simulink model "generic_src"  (Simulink 10.3)
settings: Solver=ode45  StartTime=0.0  StopTime=inf  RelTol=1e-3  EnableMultiTasking=on
undefined symbols (not defined in the file or in its folder): Area_Front, Area_Rear, ay_max_off, ay_max_on, ay_per_mu_max_off, ay_per_mu_max_on, Brake_ratio, brake_valve_ctrl_kP, cat1mode1_higher, cat1mode1_lower, cat1mode2_higher, cat1mode2_lower, cat1mode3_higher, cat1mode3_lower, cat2mode1_higher, cat2mode1_lower, cat2mode2_higher, cat2mode2_lower, cat2mode3_higher, cat2mode3_lower, delta_vel, diff_lock_fac, diff_lock_off, diff_lock_on, ESP_ctrl_kD, ESP_ctrl_kI, ESP_ctrl_kP, ESP_ctrl_restore_kI, ESP_min_throttle_fac, f_ax, f_slip, g, higherlimit_highvel, higherlimit_lowvel, highervel_fac, highervelocity_fac, InitialConditionForIntegrator, limit_acc, limit_selectlow, limit_starting, limit_vdiff, locktime_throttle, lowerlimit_highvel, lowerlimit_lowvel, lowervel_fac, lowervelocity_fac, min_throttle, MPS2KMPH, MSR_ctrl_kD, MSR_ctrl_kI, MSR_ctrl_kP, MSR_min_throttle_fac, PID_kP_sideslip, PID_kP_yawrate, RADpS2RpM, rBrake, RpM2RADpS, SH_SL_switch, sideslip_vel_corr, sidesplip_deviation_max ... (+35)
libraries: CarMaker4SL x136, simulink x55, simulink_extras x6
(part 5 of 9)

== system generic_src/CarMaker/IPG Vehicle/PowerTrain/PTControl Example/PTControl_In/CreateBus PTC BatteryLVIn ==
  In : Inport
  BusCreator : BusCreator  Inputs=8
  Demux : Demux  Outputs=8
      settings: DisplayOption=none
  Out : Outport  VectorParamsAs1DForOutWhenUnconnected=off
  wires:
  Demux/7 -> BusCreator/7  "PTC BattLVIn Temp"
  In/1 -> Demux/1
  Demux/8 -> BusCreator/8  "PTC BattLVIn TempCool_out"
  Demux/6 -> BusCreator/6  "PTC BattLVIn Pwr_max"
  Demux/1 -> BusCreator/1  "PTC BattLVIn SOC"
  Demux/3 -> BusCreator/3  "PTC BattLVIn Current"
  Demux/2 -> BusCreator/2  "PTC BattLVIn SOH"
  BusCreator/1 -> Out/1
  Demux/4 -> BusCreator/4  "PTC BattLVIn AOC"
  Demux/5 -> BusCreator/5  "PTC BattLVIn Energy"

== system generic_src/CarMaker/IPG Vehicle/PowerTrain/PTControl Example/PTControl_In/CreateBus PTC ClutchIn0 ==
  In : Inport
  BusCreator : BusCreator  Inputs=6
  Demux : Demux  Outputs=6
      settings: DisplayOption=none
  Out : Outport  VectorParamsAs1DForOutWhenUnconnected=off
  wires:
  Demux/6 -> BusCreator/6  "PTC ClutchIn0 i_TrqIn2Out"
  Demux/5 -> BusCreator/5  "PTC ClutchIn0 Trq_out"
  Demux/4 -> BusCreator/4  "PTC ClutchIn0 Trq_in"
  Demux/3 -> BusCreator/3  "PTC ClutchIn0 rotv_out"
  Demux/2 -> BusCreator/2  "PTC ClutchIn0 rotv_in"
  Demux/1 -> BusCreator/1  "PTC ClutchIn0 Pos"
  BusCreator/1 -> Out/1
  In/1 -> Demux/1

== system generic_src/CarMaker/IPG Vehicle/PowerTrain/PTControl Example/PTControl_In/CreateBus PTC ClutchIn1 ==
  In : Inport
  BusCreator : BusCreator  Inputs=6
  Demux : Demux  Outputs=6
      settings: DisplayOption=none
  Out : Outport  VectorParamsAs1DForOutWhenUnconnected=off
  wires:
  Demux/6 -> BusCreator/6  "PTC ClutchIn1 i_TrqIn2Out"
  Demux/5 -> BusCreator/5  "PTC ClutchIn1 Trq_out"
  Demux/4 -> BusCreator/4  "PTC ClutchIn1 Trq_in"
  Demux/3 -> BusCreator/3  "PTC ClutchIn1 rotv_out"
  Demux/2 -> BusCreator/2  "PTC ClutchIn1 rotv_in"
  Demux/1 -> BusCreator/1  "PTC ClutchIn1 Pos"
  BusCreator/1 -> Out/1
  In/1 -> Demux/1

== system generic_src/CarMaker/IPG Vehicle/PowerTrain/PTControl Example/PTControl_In/CreateBus PTC ClutchIn10 ==
  In : Inport
  BusCreator : BusCreator  Inputs=6
  Demux : Demux  Outputs=6
      settings: DisplayOption=none
  Out : Outport  VectorParamsAs1DForOutWhenUnconnected=off
  wires:
  Demux/6 -> BusCreator/6  "PTC ClutchIn10 i_TrqIn2Out"
  Demux/5 -> BusCreator/5  "PTC ClutchIn10 Trq_out"
  Demux/4 -> BusCreator/4  "PTC ClutchIn10 Trq_in"
  Demux/3 -> BusCreator/3  "PTC ClutchIn10 rotv_out"
  Demux/2 -> BusCreator/2  "PTC ClutchIn10 rotv_in"
  Demux/1 -> BusCreator/1  "PTC ClutchIn10 Pos"
  BusCreator/1 -> Out/1
  In/1 -> Demux/1

== system generic_src/CarMaker/IPG Vehicle/PowerTrain/PTControl Example/PTControl_In/CreateBus PTC ClutchIn11 ==
  In : Inport
  BusCreator : BusCreator  Inputs=6
  Demux : Demux  Outputs=6
      settings: DisplayOption=none
  Out : Outport  VectorParamsAs1DForOutWhenUnconnected=off
  wires:
  Demux/6 -> BusCreator/6  "PTC ClutchIn11 i_TrqIn2Out"
  Demux/5 -> BusCreator/5  "PTC ClutchIn11 Trq_out"
  Demux/4 -> BusCreator/4  "PTC ClutchIn11 Trq_in"
  Demux/3 -> BusCreator/3  "PTC ClutchIn11 rotv_out"
  Demux/2 -> BusCreator/2  "PTC ClutchIn11 rotv_in"
  Demux/1 -> BusCreator/1  "PTC ClutchIn11 Pos"
  BusCreator/1 -> Out/1
  In/1 -> Demux/1

== system generic_src/CarMaker/IPG Vehicle/PowerTrain/PTControl Example/PTControl_In/CreateBus PTC ClutchIn2 ==
  In : Inport
  BusCreator : BusCreator  Inputs=6
  Demux : Demux  Outputs=6
      settings: DisplayOption=none
  Out : Outport  VectorParamsAs1DForOutWhenUnconnected=off
  wires:
  Demux/6 -> BusCreator/6  "PTC ClutchIn2 i_TrqIn2Out"
  Demux/5 -> BusCreator/5  "PTC ClutchIn2 Trq_out"
  Demux/4 -> BusCreator/4  "PTC ClutchIn2 Trq_in"
  Demux/3 -> BusCreator/3  "PTC ClutchIn2 rotv_out"
  Demux/2 -> BusCreator/2  "PTC ClutchIn2 rotv_in"
  Demux/1 -> BusCreator/1  "PTC ClutchIn2 Pos"
  BusCreator/1 -> Out/1
  In/1 -> Demux/1

== system generic_src/CarMaker/IPG Vehicle/PowerTrain/PTControl Example/PTControl_In/CreateBus PTC ClutchIn3 ==
  In : Inport
  BusCreator : BusCreator  Inputs=6
  Demux : Demux  Outputs=6
      settings: DisplayOption=none
  Out : Outport  VectorParamsAs1DForOutWhenUnconnected=off
  wires:
  Demux/6 -> BusCreator/6  "PTC ClutchIn3 i_TrqIn2Out"
  Demux/5 -> BusCreator/5  "PTC ClutchIn3 Trq_out"
  Demux/4 -> BusCreator/4  "PTC ClutchIn3 Trq_in"
  Demux/3 -> BusCreator/3  "PTC ClutchIn3 rotv_out"
  Demux/2 -> BusCreator/2  "PTC ClutchIn3 rotv_in"
  Demux/1 -> BusCreator/1  "PTC ClutchIn3 Pos"
  BusCreator/1 -> Out/1
  In/1 -> Demux/1

== system generic_src/CarMaker/IPG Vehicle/PowerTrain/PTControl Example/PTControl_In/CreateBus PTC ClutchIn4 ==
  In : Inport
  BusCreator : BusCreator  Inputs=6
  Demux : Demux  Outputs=6
      settings: DisplayOption=none
  Out : Outport  VectorParamsAs1DForOutWhenUnconnected=off
  wires:
  Demux/6 -> BusCreator/6  "PTC ClutchIn4 i_TrqIn2Out"
  Demux/5 -> BusCreator/5  "PTC ClutchIn4 Trq_out"
  Demux/4 -> BusCreator/4  "PTC ClutchIn4 Trq_in"
  Demux/3 -> BusCreator/3  "PTC ClutchIn4 rotv_out"
  Demux/2 -> BusCreator/2  "PTC ClutchIn4 rotv_in"
  Demux/1 -> BusCreator/1  "PTC ClutchIn4 Pos"
  BusCreator/1 -> Out/1
  In/1 -> Demux/1

== system generic_src/CarMaker/IPG Vehicle/PowerTrain/PTControl Example/PTControl_In/CreateBus PTC ClutchIn5 ==
  In : Inport
  BusCreator : BusCreator  Inputs=6
  Demux : Demux  Outputs=6
      settings: DisplayOption=none
  Out : Outport  VectorParamsAs1DForOutWhenUnconnected=off
  wires:
  Demux/6 -> BusCreator/6  "PTC ClutchIn5 i_TrqIn2Out"
  Demux/5 -> BusCreator/5  "PTC ClutchIn5 Trq_out"
  Demux/4 -> BusCreator/4  "PTC ClutchIn5 Trq_in"
  Demux/3 -> BusCreator/3  "PTC ClutchIn5 rotv_out"
  Demux/2 -> BusCreator/2  "PTC ClutchIn5 rotv_in"
  Demux/1 -> BusCreator/1  "PTC ClutchIn5 Pos"
  BusCreator/1 -> Out/1
  In/1 -> Demux/1

== system generic_src/CarMaker/IPG Vehicle/PowerTrain/PTControl Example/PTControl_In/CreateBus PTC ClutchIn6 ==
  In : Inport
  BusCreator : BusCreator  Inputs=6
  Demux : Demux  Outputs=6
      settings: DisplayOption=none
  Out : Outport  VectorParamsAs1DForOutWhenUnconnected=off
  wires:
  Demux/6 -> BusCreator/6  "PTC ClutchIn6 i_TrqIn2Out"
  Demux/5 -> BusCreator/5  "PTC ClutchIn6 Trq_out"
  Demux/4 -> BusCreator/4  "PTC ClutchIn6 Trq_in"
  Demux/3 -> BusCreator/3  "PTC ClutchIn6 rotv_out"
  Demux/2 -> BusCreator/2  "PTC ClutchIn6 rotv_in"
  Demux/1 -> BusCreator/1  "PTC ClutchIn6 Pos"
  BusCreator/1 -> Out/1
  In/1 -> Demux/1

== system generic_src/CarMaker/IPG Vehicle/PowerTrain/PTControl Example/PTControl_In/CreateBus PTC ClutchIn7 ==
  In : Inport
  BusCreator : BusCreator  Inputs=6
  Demux : Demux  Outputs=6
      settings: DisplayOption=none
  Out : Outport  VectorParamsAs1DForOutWhenUnconnected=off
  wires:
  Demux/6 -> BusCreator/6  "PTC ClutchIn7 i_TrqIn2Out"
  Demux/5 -> BusCreator/5  "PTC ClutchIn7 Trq_out"
  Demux/4 -> BusCreator/4  "PTC ClutchIn7 Trq_in"
  Demux/3 -> BusCreator/3  "PTC ClutchIn7 rotv_out"
  Demux/2 -> BusCreator/2  "PTC ClutchIn7 rotv_in"
  Demux/1 -> BusCreator/1  "PTC ClutchIn7 Pos"
  BusCreator/1 -> Out/1
  In/1 -> Demux/1

== system generic_src/CarMaker/IPG Vehicle/PowerTrain/PTControl Example/PTControl_In/CreateBus PTC ClutchIn8 ==
  In : Inport
  BusCreator : BusCreator  Inputs=6
  Demux : Demux  Outputs=6
      settings: DisplayOption=none
  Out : Outport  VectorParamsAs1DForOutWhenUnconnected=off
  wires:
  Demux/6 -> BusCreator/6  "PTC ClutchIn8 i_TrqIn2Out"
  Demux/5 -> BusCreator/5  "PTC ClutchIn8 Trq_out"
  Demux/4 -> BusCreator/4  "PTC ClutchIn8 Trq_in"
  Demux/3 -> BusCreator/3  "PTC ClutchIn8 rotv_out"
  Demux/2 -> BusCreator/2  "PTC ClutchIn8 rotv_in"
  Demux/1 -> BusCreator/1  "PTC ClutchIn8 Pos"
  BusCreator/1 -> Out/1
  In/1 -> Demux/1

== system generic_src/CarMaker/IPG Vehicle/PowerTrain/PTControl Example/PTControl_In/CreateBus PTC ClutchIn9 ==
  In : Inport
  BusCreator : BusCreator  Inputs=6
  Demux : Demux  Outputs=6
      settings: DisplayOption=none
  Out : Outport  VectorParamsAs1DForOutWhenUnconnected=off
  wires:
  Demux/6 -> BusCreator/6  "PTC ClutchIn9 i_TrqIn2Out"
  Demux/5 -> BusCreator/5  "PTC ClutchIn9 Trq_out"
  Demux/4 -> BusCreator/4  "PTC ClutchIn9 Trq_in"
  Demux/3 -> BusCreator/3  "PTC ClutchIn9 rotv_out"
  Demux/2 -> BusCreator/2  "PTC ClutchIn9 rotv_in"
  Demux/1 -> BusCreator/1  "PTC ClutchIn9 Pos"
  BusCreator/1 -> Out/1
  In/1 -> Demux/1

== system generic_src/CarMaker/IPG Vehicle/PowerTrain/PTControl Example/PTControl_In/CreateBus PTC Control Units ==
  In : Inport
  BusCreator : BusCreator  Inputs=4
  Demux : Demux
      settings: DisplayOption=none
  Out : Outport  VectorParamsAs1DForOutWhenUnconnected=off
  wires:
  Demux/4 -> BusCreator/4  "PTC BCU_Status"
  Demux/3 -> BusCreator/3  "PTC TCU_Status"
  Demux/2 -> BusCreator/2  "PTC MCU_Status"
  Demux/1 -> BusCreator/1  "PTC ECU_Status"
  BusCreator/1 -> Out/1
  In/1 -> Demux/1

== system generic_src/CarMaker/IPG Vehicle/PowerTrain/PTControl Example/PTControl_In/CreateBus PTC DriveSrcIn ==
  In : Inport
  BusCreator : BusCreator  Inputs=4
  Demux : Demux
      settings: DisplayOption=none
  Out : Outport  VectorParamsAs1DForOutWhenUnconnected=off
  wires:
  Demux/4 -> BusCreator/4  "PTC DriveSrcIn_d3 Trq_DriveSrc_trg"
  Demux/3 -> BusCreator/3  "PTC DriveSrcIn_d2 Trq_DriveSrc_trg"
  Demux/2 -> BusCreator/2  "PTC DriveSrcIn_d1 Trq_DriveSrc_trg"
  Demux/1 -> BusCreator/1  "PTC DriveSrcIn_d0 Trq_DriveSrc_trg"
  BusCreator/1 -> Out/1
  In/1 -> Demux/1

== system generic_src/CarMaker/IPG Vehicle/PowerTrain/PTControl Example/PTControl_In/CreateBus PTC EngineIn ==
  In : Inport
  BusCreator : BusCreator  Inputs=7
  Demux : Demux  Outputs=7
      settings: DisplayOption=none
  Out : Outport  VectorParamsAs1DForOutWhenUnconnected=off
  wires:
  Demux/7 -> BusCreator/7  "PTC EngineIn FuelFlow"
  Demux/6 -> BusCreator/6  "PTC EngineIn TrqOpt"
  Demux/5 -> BusCreator/5  "PTC EngineIn TrqFull"
  Demux/4 -> BusCreator/4  "PTC EngineIn TrqDrag"
  Demux/3 -> BusCreator/3  "PTC EngineIn Trq"
  Demux/2 -> BusCreator/2  "PTC EngineIn rotv"
  Demux/1 -> BusCreator/1  "PTC EngineIn Engine_on"
  BusCreator/1 -> Out/1
  In/1 -> Demux/1

== system generic_src/CarMaker/IPG Vehicle/PowerTrain/PTControl Example/PTControl_In/CreateBus PTC GearboxIn0 ==
  In : Inport
  BusCreator : BusCreator  Inputs=20
  Demux : Demux  Outputs=20
      settings: DisplayOption=none
  Out : Outport  VectorParamsAs1DForOutWhenUnconnected=off
  wires:
  Demux/20 -> BusCreator/20  "PTC GearboxIn0 Clutch_dis i_TrqIn2Out"
  Demux/19 -> BusCreator/19  "PTC GearboxIn0 Clutch_dis Trq_out"
  Demux/18 -> BusCreator/18  "PTC GearboxIn0 Clutch_dis Trq_in"
  Demux/17 -> BusCreator/17  "PTC GearboxIn0 Clutch_dis rotv_out"
  Demux/16 -> BusCreator/16  "PTC GearboxIn0 Clutch_dis rotv_in"
  Demux/15 -> BusCreator/15  "PTC GearboxIn0 Clutch_dis Pos"
  Demux/14 -> BusCreator/14  "PTC GearboxIn0 Clutch i_TrqIn2Out"
  Demux/13 -> BusCreator/13  "PTC GearboxIn0 Clutch Trq_out"
  Demux/12 -> BusCreator/12  "PTC GearboxIn0 Clutch Trq_in"
  Demux/11 -> BusCreator/11  "PTC GearboxIn0 Clutch rotv_out"
  Demux/10 -> BusCreator/10  "PTC GearboxIn0 Clutch rotv_in"
  Demux/9 -> BusCreator/9  "PTC GearboxIn0 Clutch Pos"
  Demux/8 -> BusCreator/8  "PTC GearboxIn0 Trq_out"
  Demux/7 -> BusCreator/7  "PTC GearboxIn0 Trq_in"
  Demux/6 -> BusCreator/6  "PTC GearboxIn0 rotv_out"
  Demux/5 -> BusCreator/5  "PTC GearboxIn0 rotv_in"
  Demux/4 -> BusCreator/4  "PTC GearboxIn0 i"
  Demux/3 -> BusCreator/3  "PTC GearboxIn0 Trq_DriveSrc_trg"
  Demux/2 -> BusCreator/2  "PTC GearboxIn0 GearNo_dis"
  Demux/1 -> BusCreator/1  "PTC GearboxIn0 GearNo"
  BusCreator/1 -> Out/1
  In/1 -> Demux/1

== system generic_src/CarMaker/IPG Vehicle/PowerTrain/PTControl Example/PTControl_In/CreateBus PTC GearboxIn1 ==
  In : Inport
  BusCreator : BusCreator  Inputs=20
  Demux : Demux  Outputs=20
      settings: DisplayOption=none
  Out : Outport  VectorParamsAs1DForOutWhenUnconnected=off
  wires:
  Demux/20 -> BusCreator/20  "PTC GearboxIn1 Clutch_dis i_TrqIn2Out"
  Demux/19 -> BusCreator/19  "PTC GearboxIn1 Clutch_dis Trq_out"
  Demux/18 -> BusCreator/18  "PTC GearboxIn1 Clutch_dis Trq_in"
  Demux/17 -> BusCreator/17  "PTC GearboxIn1 Clutch_dis rotv_out"
  Demux/16 -> BusCreator/16  "PTC GearboxIn1 Clutch_dis rotv_in"
  Demux/15 -> BusCreator/15  "PTC GearboxIn1 Clutch_dis Pos"
  Demux/14 -> BusCreator/14  "PTC GearboxIn1 Clutch i_TrqIn2Out"
  Demux/13 -> BusCreator/13  "PTC GearboxIn1 Clutch Trq_out"
  Demux/12 -> BusCreator/12  "PTC GearboxIn1 Clutch Trq_in"
  Demux/11 -> BusCreator/11  "PTC GearboxIn1 Clutch rotv_out"
  Demux/10 -> BusCreator/10  "PTC GearboxIn1 Clutch rotv_in"
  Demux/9 -> BusCreator/9  "PTC GearboxIn1 Clutch Pos"
  Demux/8 -> BusCreator/8  "PTC GearboxIn1 Trq_out"
  Demux/7 -> BusCreator/7  "PTC GearboxIn1 Trq_in"
  Demux/6 -> BusCreator/6  "PTC GearboxIn1 rotv_out"
  Demux/5 -> BusCreator/5  "PTC GearboxIn1 rotv_in"
  Demux/4 -> BusCreator/4  "PTC GearboxIn1 i"
  Demux/3 -> BusCreator/3  "PTC GearboxIn1 Trq_DriveSrc_trg"
  Demux/2 -> BusCreator/2  "PTC GearboxIn1 GearNo_dis"
  Demux/1 -> BusCreator/1  "PTC GearboxIn1 GearNo"
  BusCreator/1 -> Out/1
  In/1 -> Demux/1

== system generic_src/CarMaker/IPG Vehicle/PowerTrain/PTControl Example/PTControl_In/CreateBus PTC GearboxIn10 ==
  In : Inport
  BusCreator : BusCreator  Inputs=20
  Demux : Demux  Outputs=20
      settings: DisplayOption=none
  Out : Outport  VectorParamsAs1DForOutWhenUnconnected=off
  wires:
  Demux/20 -> BusCreator/20  "PTC GearboxIn10 Clutch_dis i_TrqIn2Out"
  Demux/19 -> BusCreator/19  "PTC GearboxIn10 Clutch_dis Trq_out"
  Demux/18 -> BusCreator/18  "PTC GearboxIn10 Clutch_dis Trq_in"
  Demux/17 -> BusCreator/17  "PTC GearboxIn10 Clutch_dis rotv_out"
  Demux/16 -> BusCreator/16  "PTC GearboxIn10 Clutch_dis rotv_in"
  Demux/15 -> BusCreator/15  "PTC GearboxIn10 Clutch_dis Pos"
  Demux/14 -> BusCreator/14  "PTC GearboxIn10 Clutch i_TrqIn2Out"
  Demux/13 -> BusCreator/13  "PTC GearboxIn10 Clutch Trq_out"
  Demux/12 -> BusCreator/12  "PTC GearboxIn10 Clutch Trq_in"
  Demux/11 -> BusCreator/11  "PTC GearboxIn10 Clutch rotv_out"
  Demux/10 -> BusCreator/10  "PTC GearboxIn10 Clutch rotv_in"
  Demux/9 -> BusCreator/9  "PTC GearboxIn10 Clutch Pos"
  Demux/8 -> BusCreator/8  "PTC GearboxIn10 Trq_out"
  Demux/7 -> BusCreator/7  "PTC GearboxIn10 Trq_in"
  Demux/6 -> BusCreator/6  "PTC GearboxIn10 rotv_out"
  Demux/5 -> BusCreator/5  "PTC GearboxIn10 rotv_in"
  Demux/4 -> BusCreator/4  "PTC GearboxIn10 i"
  Demux/3 -> BusCreator/3  "PTC GearboxIn10 Trq_DriveSrc_trg"
  Demux/2 -> BusCreator/2  "PTC GearboxIn10 GearNo_dis"
  Demux/1 -> BusCreator/1  "PTC GearboxIn10 GearNo"
  BusCreator/1 -> Out/1
  In/1 -> Demux/1

== system generic_src/CarMaker/IPG Vehicle/PowerTrain/PTControl Example/PTControl_In/CreateBus PTC GearboxIn11 ==
  In : Inport
  BusCreator : BusCreator  Inputs=20
  Demux : Demux  Outputs=20
      settings: DisplayOption=none
  Out : Outport  VectorParamsAs1DForOutWhenUnconnected=off
  wires:
  Demux/20 -> BusCreator/20  "PTC GearboxIn11 Clutch_dis i_TrqIn2Out"
  Demux/19 -> BusCreator/19  "PTC GearboxIn11 Clutch_dis Trq_out"
  Demux/18 -> BusCreator/18  "PTC GearboxIn11 Clutch_dis Trq_in"
  Demux/17 -> BusCreator/17  "PTC GearboxIn11 Clutch_dis rotv_out"
  Demux/16 -> BusCreator/16  "PTC GearboxIn11 Clutch_dis rotv_in"
  Demux/15 -> BusCreator/15  "PTC GearboxIn11 Clutch_dis Pos"
  Demux/14 -> BusCreator/14  "PTC GearboxIn11 Clutch i_TrqIn2Out"
  Demux/13 -> BusCreator/13  "PTC GearboxIn11 Clutch Trq_out"
  Demux/12 -> BusCreator/12  "PTC GearboxIn11 Clutch Trq_in"
  Demux/11 -> BusCreator/11  "PTC GearboxIn11 Clutch rotv_out"
  Demux/10 -> BusCreator/10  "PTC GearboxIn11 Clutch rotv_in"
  Demux/9 -> BusCreator/9  "PTC GearboxIn11 Clutch Pos"
  Demux/8 -> BusCreator/8  "PTC GearboxIn11 Trq_out"
  Demux/7 -> BusCreator/7  "PTC GearboxIn11 Trq_in"
  Demux/6 -> BusCreator/6  "PTC GearboxIn11 rotv_out"
  Demux/5 -> BusCreator/5  "PTC GearboxIn11 rotv_in"
  Demux/4 -> BusCreator/4  "PTC GearboxIn11 i"
  Demux/3 -> BusCreator/3  "PTC GearboxIn11 Trq_DriveSrc_trg"
  Demux/2 -> BusCreator/2  "PTC GearboxIn11 GearNo_dis"
  Demux/1 -> BusCreator/1  "PTC GearboxIn11 GearNo"
  BusCreator/1 -> Out/1
  In/1 -> Demux/1

== system generic_src/CarMaker/IPG Vehicle/PowerTrain/PTControl Example/PTControl_In/CreateBus PTC GearboxIn2 ==
  In : Inport
  BusCreator : BusCreator  Inputs=20
  Demux : Demux  Outputs=20
      settings: DisplayOption=none
  Out : Outport  VectorParamsAs1DForOutWhenUnconnected=off
  wires:
  Demux/20 -> BusCreator/20  "PTC GearboxIn2 Clutch_dis i_TrqIn2Out"
  Demux/19 -> BusCreator/19  "PTC GearboxIn2 Clutch_dis Trq_out"
  Demux/18 -> BusCreator/18  "PTC GearboxIn2 Clutch_dis Trq_in"
  Demux/17 -> BusCreator/17  "PTC GearboxIn2 Clutch_dis rotv_out"
  Demux/16 -> BusCreator/16  "PTC GearboxIn2 Clutch_dis rotv_in"
  Demux/15 -> BusCreator/15  "PTC GearboxIn2 Clutch_dis Pos"
  Demux/14 -> BusCreator/14  "PTC GearboxIn2 Clutch i_TrqIn2Out"
  Demux/13 -> BusCreator/13  "PTC GearboxIn2 Clutch Trq_out"
  Demux/12 -> BusCreator/12  "PTC GearboxIn2 Clutch Trq_in"
  Demux/11 -> BusCreator/11  "PTC GearbxIn2 Clutch rotv_out"
  Demux/10 -> BusCreator/10  "PTC GearboxIn2 Clutch rotv_in"
  Demux/9 -> BusCreator/9  "PTC GearboxIn2 Clutch Pos"
  Demux/8 -> BusCreator/8  "PTC GearboxIn2 Trq_out"
  Demux/7 -> BusCreator/7  "PTC GearboxIn2 Trq_in"
  Demux/6 -> BusCreator/6  "PTC GearboxIn2 rotv_out"
  Demux/5 -> BusCreator/5  "PTC GearboxIn2 rotv_in"
  Demux/4 -> BusCreator/4  "PTC GearboxIn2 i"
  Demux/3 -> BusCreator/3  "PTC GearboxIn2 Trq_DriveSrc_trg"
  Demux/2 -> BusCreator/2  "PTC GearboxIn2 GearNo_dis"
  Demux/1 -> BusCreator/1  "PTC GearboxIn2 GearNo"
  BusCreator/1 -> Out/1
  In/1 -> Demux/1

== system generic_src/CarMaker/IPG Vehicle/PowerTrain/PTControl Example/PTControl_In/CreateBus PTC GearboxIn3 ==
  In : Inport
  BusCreator : BusCreator  Inputs=20
  Demux : Demux  Outputs=20
      settings: DisplayOption=none
  Out : Outport  VectorParamsAs1DForOutWhenUnconnected=off
  wires:
  Demux/20 -> BusCreator/20  "PTC GearboxIn3 Clutch_dis i_TrqIn2Out"
  Demux/19 -> BusCreator/19  "PTC GearboxIn3 Clutch_dis Trq_out"
  Demux/18 -> BusCreator/18  "PTC GearboxIn3 Clutch_dis Trq_in"
  Demux/17 -> BusCreator/17  "PTC GearboxIn3 Clutch_dis rotv_out"
  Demux/16 -> BusCreator/16  "PTC GearboxIn3 Clutch_dis rotv_in"
  Demux/15 -> BusCreator/15  "PTC GearboxIn3 Clutch_dis Pos"
  Demux/14 -> BusCreator/14  "PTC GearboxIn3 Clutch i_TrqIn2Out"
  Demux/13 -> BusCreator/13  "PTC GearboxIn3 Clutch Trq_out"
  Demux/12 -> BusCreator/12  "PTC GearboxIn3 Clutch Trq_in"
  Demux/11 -> BusCreator/11  "PTC GearboxIn3 Clutch rotv_out"
  Demux/10 -> BusCreator/10  "PTC GearboxIn3 Clutch rotv_in"
  Demux/9 -> BusCreator/9  "PTC GearboxIn3 Clutch Pos"
  Demux/8 -> BusCreator/8  "PTC GearboxIn3 Trq_out"
  Demux/7 -> BusCreator/7  "PTC GearboxIn3 Trq_in"
  Demux/6 -> BusCreator/6  "PTC GearboxIn3 rotv_out"
  Demux/5 -> BusCreator/5  "PTC GearboxIn3 rotv_in"
  Demux/4 -> BusCreator/4  "PTC GearboxIn3 i"
  Demux/3 -> BusCreator/3  "PTC GearboxIn3 Trq_DriveSrc_trg"
  Demux/2 -> BusCreator/2  "PTC GearboxIn3 GearNo_dis"
  Demux/1 -> BusCreator/1  "PTC GearboxIn3 GearNo"
  BusCreator/1 -> Out/1
  In/1 -> Demux/1

== system generic_src/CarMaker/IPG Vehicle/PowerTrain/PTControl Example/PTControl_In/CreateBus PTC GearboxIn4 ==
  In : Inport
  BusCreator : BusCreator  Inputs=20
  Demux : Demux  Outputs=20
      settings: DisplayOption=none
  Out : Outport  VectorParamsAs1DForOutWhenUnconnected=off
  wires:
  Demux/20 -> BusCreator/20  "PTC GearboxIn4 Clutch_dis i_TrqIn2Out"
  Demux/19 -> BusCreator/19  "PTC GearboxIn4 Clutch_dis Trq_out"
  Demux/18 -> BusCreator/18  "PTC GearboxIn4 Clutch_dis Trq_in"
  Demux/17 -> BusCreator/17  "PTC GearboxIn4 Clutch_dis rotv_out"
  Demux/16 -> BusCreator/16  "PTC GearboxIn4 Clutch_dis rotv_in"
  Demux/15 -> BusCreator/15  "PTC GearboxIn4 Clutch_dis Pos"
  Demux/14 -> BusCreator/14  "PTC GearboxIn4 Clutch i_TrqIn2Out"
  Demux/13 -> BusCreator/13  "PTC GearboxIn4 Clutch Trq_out"
  Demux/12 -> BusCreator/12  "PTC GearboxIn4 Clutch Trq_in"
  Demux/11 -> BusCreator/11  "PTC GearboxIn4 Clutch rotv_out"
  Demux/10 -> BusCreator/10  "PTC GearboxIn4 Clutch rotv_in"
  Demux/9 -> BusCreator/9  "PTC GearboxIn4 Clutch Pos"
  Demux/8 -> BusCreator/8  "PTC GearboxIn4 Trq_out"
  Demux/7 -> BusCreator/7  "PTC GearboxIn4 Trq_in"
  Demux/6 -> BusCreator/6  "PTC GearboxIn4 rotv_out"
  Demux/5 -> BusCreator/5  "PTC GearboxIn4 rotv_in"
  Demux/4 -> BusCreator/4  "PTC GearboxIn4 i"
  Demux/3 -> BusCreator/3  "PTC GearboxIn4 Trq_DriveSrc_trg"
  Demux/2 -> BusCreator/2  "PTC GearboxIn4 GearNo_dis"
  Demux/1 -> BusCreator/1  "PTC GearboxIn4 GearNo"
  BusCreator/1 -> Out/1
  In/1 -> Demux/1

== system generic_src/CarMaker/IPG Vehicle/PowerTrain/PTControl Example/PTControl_In/CreateBus PTC GearboxIn5 ==
  In : Inport
  BusCreator : BusCreator  Inputs=20
  Demux : Demux  Outputs=20
      settings: DisplayOption=none
  Out : Outport  VectorParamsAs1DForOutWhenUnconnected=off
  wires:
  Demux/20 -> BusCreator/20  "PTC GearboxIn5 Clutch_dis i_TrqIn2Out"
  Demux/19 -> BusCreator/19  "PTC GearboxIn5 Clutch_dis Trq_out"
  Demux/18 -> BusCreator/18  "PTC GearboxIn5 Clutch_dis Trq_in"
  Demux/17 -> BusCreator/17  "PTC GearboxIn5 Clutch_dis rotv_out"
  Demux/16 -> BusCreator/16  "PTC GearboxIn5 Clutch_dis rotv_in"
  Demux/15 -> BusCreator/15  "PTC GearboxIn5 Clutch_dis Pos"
  Demux/14 -> BusCreator/14  "PTC GearboxIn5 Clutch i_TrqIn2Out"
  Demux/13 -> BusCreator/13  "PTC GearboxIn5 Clutch Trq_out"
  Demux/12 -> BusCreator/12  "PTC GearboxIn5 Clutch Trq_in"
  Demux/11 -> BusCreator/11  "PTC GearboxIn5 Clutch rotv_out"
  Demux/10 -> BusCreator/10  "PTC GearboxIn5 Clutch rotv_in"
  Demux/9 -> BusCreator/9  "PTC GearboxIn5 Clutch Pos"
  Demux/8 -> BusCreator/8  "PTC GearboxIn5 Trq_out"
  Demux/7 -> BusCreator/7  "PTC GearboxIn5 Trq_in"
  Demux/6 -> BusCreator/6  "PTC GearboxIn5 rotv_out"
  Demux/5 -> BusCreator/5  "PTC GearboxIn5 rotv_in"
  Demux/4 -> BusCreator/4  "PTC GearboxIn5 i"
  Demux/3 -> BusCreator/3  "PTC GearboxIn5 Trq_DriveSrc_trg"
  Demux/2 -> BusCreator/2  "PTC GearboxIn5 GearNo_dis"
  Demux/1 -> BusCreator/1  "PTC GearboxIn5 GearNo"
  BusCreator/1 -> Out/1
  In/1 -> Demux/1

== system generic_src/CarMaker/IPG Vehicle/PowerTrain/PTControl Example/PTControl_In/CreateBus PTC GearboxIn6 ==
  In : Inport
  BusCreator : BusCreator  Inputs=20
  Demux : Demux  Outputs=20
      settings: DisplayOption=none
  Out : Outport  VectorParamsAs1DForOutWhenUnconnected=off
  wires:
  Demux/20 -> BusCreator/20  "PTC GearboxIn6 Clutch_dis i_TrqIn2Out"
  Demux/19 -> BusCreator/19  "PTC GearboxIn6 Clutch_dis Trq_out"
  Demux/18 -> BusCreator/18  "PTC GearboxIn6 Clutch_dis Trq_in"
  Demux/17 -> BusCreator/17  "PTC GearboxIn6 Clutch_dis rotv_out"
  Demux/16 -> BusCreator/16  "PTC GearboxIn6 Clutch_dis rotv_in"
  Demux/15 -> BusCreator/15  "PTC GearboxIn6 Clutch_dis Pos"
  Demux/14 -> BusCreator/14  "PTC GearboxIn6 Clutch i_TrqIn2Out"
  Demux/13 -> BusCreator/13  "PTC GearboxIn6 Clutch Trq_out"
  Demux/12 -> BusCreator/12  "PTC GearboxIn6 Clutch Trq_in"
  Demux/11 -> BusCreator/11  "PTC GearboxIn6 Clutch rotv_out"
  Demux/10 -> BusCreator/10  "PTC GearboxIn6 Clutch rotv_in"
  Demux/9 -> BusCreator/9  "PTC GearboxIn6 Clutch Pos"
  Demux/8 -> BusCreator/8  "PTC GearboxIn6 Trq_out"
  Demux/7 -> BusCreator/7  "PTC GearboxIn6 Trq_in"
  Demux/6 -> BusCreator/6  "PTC GearboxIn6 rotv_out"
  Demux/5 -> BusCreator/5  "PTC GearboxIn6 rotv_in"
  Demux/4 -> BusCreator/4  "PTC GearboxIn6 i"
  Demux/3 -> BusCreator/3  "PTC GearboxIn6 Trq_DriveSrc_trg"
  Demux/2 -> BusCreator/2  "PTC GearboxIn6 GearNo_dis"
  Demux/1 -> BusCreator/1  "PTC GearboxIn6 GearNo"
  BusCreator/1 -> Out/1
  In/1 -> Demux/1

== system generic_src/CarMaker/IPG Vehicle/PowerTrain/PTControl Example/PTControl_In/CreateBus PTC GearboxIn7 ==
  In : Inport
  BusCreator : BusCreator  Inputs=20
  Demux : Demux  Outputs=20
      settings: DisplayOption=none
  Out : Outport  VectorParamsAs1DForOutWhenUnconnected=off
  wires:
  Demux/20 -> BusCreator/20  "PTC GearboxIn7 Clutch_dis i_TrqIn2Out"
  Demux/19 -> BusCreator/19  "PTC GearboxIn7 Clutch_dis Trq_out"
  Demux/18 -> BusCreator/18  "PTC GearboxIn7 Clutch_dis Trq_in"
  Demux/17 -> BusCreator/17  "PTC GearboxIn7 Clutch_dis rotv_out"
  Demux/16 -> BusCreator/16  "PTC GearboxIn7 Clutch_dis rotv_in"
  Demux/15 -> BusCreator/15  "PTC GearboxIn7 Clutch_dis Pos"
  Demux/14 -> BusCreator/14  "PTC GearboxIn7 Clutch i_TrqIn2Out"
  Demux/13 -> BusCreator/13  "PTC GearboxIn7 Clutch Trq_out"
  Demux/12 -> BusCreator/12  "PTC GearboxIn7 Clutch Trq_in"
  Demux/11 -> BusCreator/11  "PTC GearboxIn7 Clutch rotv_out"
  Demux/10 -> BusCreator/10  "PTC GearboxIn7 Clutch rotv_in"
  Demux/9 -> BusCreator/9  "PTC GearboxIn7 Clutch Pos"
  Demux/8 -> BusCreator/8  "PTC GearboxIn7 Trq_out"
  Demux/7 -> BusCreator/7  "PTC GearboxIn7 Trq_in"
  Demux/6 -> BusCreator/6  "PTC GearboxIn7 rotv_out"
  Demux/5 -> BusCreator/5  "PTC GearboxIn7 rotv_in"
  Demux/4 -> BusCreator/4  "PTC GearboxIn7 i"
  Demux/3 -> BusCreator/3  "PTC GearboxIn7 Trq_DriveSrc_trg"
  Demux/2 -> BusCreator/2  "PTC GearboxIn7 GearNo_dis"
  Demux/1 -> BusCreator/1  "PTC GearboxIn7 GearNo"
  BusCreator/1 -> Out/1
  In/1 -> Demux/1

== system generic_src/CarMaker/IPG Vehicle/PowerTrain/PTControl Example/PTControl_In/CreateBus PTC GearboxIn8 ==
  In : Inport
  BusCreator : BusCreator  Inputs=20
  Demux : Demux  Outputs=20
      settings: DisplayOption=none
  Out : Outport  VectorParamsAs1DForOutWhenUnconnected=off
  wires:
  Demux/20 -> BusCreator/20  "PTC GearboxIn8 Clutch_dis i_TrqIn2Out"
  Demux/19 -> BusCreator/19  "PTC GearboxIn8 Clutch_dis Trq_out"
  Demux/18 -> BusCreator/18  "PTC GearboxIn8 Clutch_dis Trq_in"
  Demux/17 -> BusCreator/17  "PTC GearboxIn8 Clutch_dis rotv_out"
  Demux/16 -> BusCreator/16  "PTC GearboxIn8 Clutch_dis rotv_in"
  Demux/15 -> BusCreator/15  "PTC GearboxIn8 Clutch_dis Pos"
  Demux/14 -> BusCreator/14  "PTC GearboxIn8 Clutch i_TrqIn2Out"
  Demux/13 -> BusCreator/13  "PTC GearboxIn8 Clutch Trq_out"
  Demux/12 -> BusCreator/12  "PTC GearboxIn8 Clutch Trq_in"
  Demux/11 -> BusCreator/11  "PTC GearboxIn8 Clutch rotv_out"
  Demux/10 -> BusCreator/10  "PTC GearboxIn8 Clutch rotv_in"
  Demux/9 -> BusCreator/9  "PTC GearboxIn8 Clutch Pos"
  Demux/8 -> BusCreator/8  "PTC GearboxIn8 Trq_out"
  Demux/7 -> BusCreator/7  "PTC GearboxIn8 Trq_in"
  Demux/6 -> BusCreator/6  "PTC GearboxIn8 rotv_out"
  Demux/5 -> BusCreator/5  "PTC GearboxIn8 rotv_in"
  Demux/4 -> BusCreator/4  "PTC GearboxIn8 i"
  Demux/3 -> BusCreator/3  "PTC GearboxIn8 Trq_DriveSrc_trg"
  Demux/2 -> BusCreator/2  "PTC GearboxIn8 GearNo_dis"
  Demux/1 -> BusCreator/1  "PTC GearboxIn8 GearNo"
  BusCreator/1 -> Out/1
  In/1 -> Demux/1

== system generic_src/CarMaker/IPG Vehicle/PowerTrain/PTControl Example/PTControl_In/CreateBus PTC GearboxIn9 ==
  In : Inport
  BusCreator : BusCreator  Inputs=20
  Demux : Demux  Outputs=20
      settings: DisplayOption=none
  Out : Outport  VectorParamsAs1DForOutWhenUnconnected=off
  wires:
  Demux/20 -> BusCreator/20  "PTC GearboxIn9 Clutch_dis i_TrqIn2Out"
  Demux/19 -> BusCreator/19  "PTC GearboxIn9 Clutch_dis Trq_out"
  Demux/18 -> BusCreator/18  "PTC GearboxIn9 Clutch_dis Trq_in"
  Demux/17 -> BusCreator/17  "PTC GearboxIn9 Clutch_dis rotv_out"
  Demux/16 -> BusCreator/16  "PTC GearboxIn9 Clutch_dis rotv_in"
  Demux/15 -> BusCreator/15  "PTC GearboxIn9 Clutch_dis Pos"
  Demux/14 -> BusCreator/14  "PTC GearboxIn9 Clutch i_TrqIn2Out"
  Demux/13 -> BusCreator/13  "PTC GearboxIn9 Clutch Trq_out"
  Demux/12 -> BusCreator/12  "PTC GearboxIn9 Clutch Trq_in"
  Demux/11 -> BusCreator/11  "PTC GearboxIn9 Clutch rotv_out"
  Demux/10 -> BusCreator/10  "PTC GearboxIn9 Clutch rotv_in"
  Demux/9 -> BusCreator/9  "PTC GearboxIn9 Clutch Pos"
  Demux/8 -> BusCreator/8  "PTC GearboxIn9 Trq_out"
  Demux/7 -> BusCreator/7  "PTC GearboxIn9 Trq_in"
  Demux/6 -> BusCreator/6  "PTC GearboxIn9 rotv_out"
  Demux/5 -> BusCreator/5  "PTC GearboxIn9 rotv_in"
  Demux/4 -> BusCreator/4  "PTC GearboxIn9 i"
  Demux/3 -> BusCreator/3  "PTC GearboxIn9 Trq_DriveSrc_trg"
  Demux/2 -> BusCreator/2  "PTC GearboxIn9 GearNo_dis"
  Demux/1 -> BusCreator/1  "PTC GearboxIn9 GearNo"
  BusCreator/1 -> Out/1
  In/1 -> Demux/1

== system generic_src/CarMaker/IPG Vehicle/PowerTrain/PTControl Example/PTControl_In/CreateBus PTC ISGIn ==
  In : Inport
  BusCreator : BusCreator  Inputs=9
  Demux : Demux  Outputs=9
      settings: DisplayOption=none
  Out : Outport  VectorParamsAs1DForOutWhenUnconnected=off
  wires:
  Demux/9 -> BusCreator/9  "PTC ISGIn i_M2W_RR"
  Demux/8 -> BusCreator/8  "PTC ISGIn i_M2W_RL"
  Demux/7 -> BusCreator/7  "PTC ISGIn i_M2W_FR"
  Demux/6 -> BusCreator/6  "PTC ISGIn i_M2W_FL"
  Demux/5 -> BusCreator/5  "PTC ISGIn PwrElec"
  Demux/4 -> BusCreator/4  "PTC ISGIn TrqGen_max"
  Demux/3 -> BusCreator/3  "PTC ISGIn TrqMot_max"
  Demux/2 -> BusCreator/2  "PTC ISGIn Trq"
  Demux/1 -> BusCreator/1  "PTC ISGIn rotv"
  BusCreator/1 -> Out/1
  In/1 -> Demux/1

== system generic_src/CarMaker/IPG Vehicle/PowerTrain/PTControl Example/PTControl_In/CreateBus PTC MotorIn0 ==
  In : Inport
  BusCreator : BusCreator  Inputs=9
  Demux : Demux  Outputs=9
      settings: DisplayOption=none
  Out : Outport  VectorParamsAs1DForOutWhenUnconnected=off
  wires:
  Demux/9 -> BusCreator/9  "PTC MotorIn0 i_M2W_RR"
  Demux/8 -> BusCreator/8  "PTC MotorIn0 i_M2W_RL"
  Demux/7 -> BusCreator/7  "PTC MotorIn0 i_M2W_FR"
  Demux/6 -> BusCreator/6  "PTC MotorIn0 i_M2W_FL"
  Demux/5 -> BusCreator/5  "PTC MotorIn0 PwrElec"
  Demux/4 -> BusCreator/4  "PTC MotorIn0 TrqGen_max"
  Demux/3 -> BusCreator/3  "PTC MotorIn0 TrqMot_max"
  Demux/2 -> BusCreator/2  "PTC MotorIn0 Trq"
  Demux/1 -> BusCreator/1  "PTC MotorIn0 rotv"
  BusCreator/1 -> Out/1
  In/1 -> Demux/1

== system generic_src/CarMaker/IPG Vehicle/PowerTrain/PTControl Example/PTControl_In/CreateBus PTC MotorIn1 ==
  In : Inport
  BusCreator : BusCreator  Inputs=9
  Demux : Demux  Outputs=9
      settings: DisplayOption=none
  Out : Outport  VectorParamsAs1DForOutWhenUnconnected=off
  wires:
  Demux/9 -> BusCreator/9  "PTC MotorIn1 i_M2W_RR"
  Demux/8 -> BusCreator/8  "PTC MotorIn1 i_M2W_RL"
  Demux/7 -> BusCreator/7  "PTC MotorIn1 i_M2W_FR"
  Demux/6 -> BusCreator/6  "PTC MotorIn1 i_M2W_FL"
  Demux/5 -> BusCreator/5  "PTC MotorIn1 PwrElec"
  Demux/4 -> BusCreator/4  "PTC MotorIn1 TrqGen_max"
  Demux/3 -> BusCreator/3  "PTC MotorIn1 TrqMot_max"
  Demux/2 -> BusCreator/2  "PTC MotorIn1 Trq"
  Demux/1 -> BusCreator/1  "PTC MotorIn1 rotv"
  BusCreator/1 -> Out/1
  In/1 -> Demux/1

== system generic_src/CarMaker/IPG Vehicle/PowerTrain/PTControl Example/PTControl_In/CreateBus PTC MotorIn10 ==
  In : Inport
  BusCreator : BusCreator  Inputs=9
  Demux : Demux  Outputs=9
      settings: DisplayOption=none
  Out : Outport  VectorParamsAs1DForOutWhenUnconnected=off
  wires:
  Demux/9 -> BusCreator/9  "PTC MotorIn10 i_M2W_RR"
  Demux/8 -> BusCreator/8  "PTC MotorIn10 i_M2W_RL"
  Demux/7 -> BusCreator/7  "PTC MotorIn10 i_M2W_FR"
  Demux/6 -> BusCreator/6  "PTC MotorIn10 i_M2W_FL"
  Demux/5 -> BusCreator/5  "PTC MotorIn10 PwrElec"
  Demux/4 -> BusCreator/4  "PTC MotorIn10 TrqGen_max"
  Demux/3 -> BusCreator/3  "PTC MotorIn10 TrqMot_max"
  Demux/2 -> BusCreator/2  "PTC MotorIn10 Trq"
  Demux/1 -> BusCreator/1  "PTC MotorIn10 rotv"
  BusCreator/1 -> Out/1
  In/1 -> Demux/1

== system generic_src/CarMaker/IPG Vehicle/PowerTrain/PTControl Example/PTControl_In/CreateBus PTC MotorIn11 ==
  In : Inport
  BusCreator : BusCreator  Inputs=9
  Demux : Demux  Outputs=9
      settings: DisplayOption=none
  Out : Outport  VectorParamsAs1DForOutWhenUnconnected=off
  wires:
  Demux/9 -> BusCreator/9  "PTC MotorIn11 i_M2W_RR"
  Demux/8 -> BusCreator/8  "PTC MotorIn11 i_M2W_RL"
  Demux/7 -> BusCreator/7  "PTC MotorIn11 i_M2W_FR"
  Demux/6 -> BusCreator/6  "PTC MotorIn11 i_M2W_FL"
  Demux/5 -> BusCreator/5  "PTC MotorIn11 PwrElec"
  Demux/4 -> BusCreator/4  "PTC MotorIn11 TrqGen_max"
  Demux/3 -> BusCreator/3  "PTC MotorIn11 TrqMot_max"
  Demux/2 -> BusCreator/2  "PTC MotorIn11 Trq"
  Demux/1 -> BusCreator/1  "PTC MotorIn11 rotv"
  BusCreator/1 -> Out/1
  In/1 -> Demux/1

== system generic_src/CarMaker/IPG Vehicle/PowerTrain/PTControl Example/PTControl_In/CreateBus PTC MotorIn2 ==
  In : Inport
  BusCreator : BusCreator  Inputs=9
  Demux : Demux  Outputs=9
      settings: DisplayOption=none
  Out : Outport  VectorParamsAs1DForOutWhenUnconnected=off
  wires:
  Demux/9 -> BusCreator/9  "PTC MotorIn2 i_M2W_RR"
  Demux/8 -> BusCreator/8  "PTC MotorIn2 i_M2W_RL"
  Demux/7 -> BusCreator/7  "PTC MotorIn2 i_M2W_FR"
  Demux/6 -> BusCreator/6  "PTC MotorIn2 i_M2W_FL"
  Demux/5 -> BusCreator/5  "PTC MotorIn2 PwrElec"
  Demux/4 -> BusCreator/4  "PTC MotorIn2 TrqGen_max"
  Demux/3 -> BusCreator/3  "PTC MotorIn2 TrqMot_max"
  Demux/2 -> BusCreator/2  "PTC MotorIn2 Trq"
  Demux/1 -> BusCreator/1  "PTC MotorIn2 rotv"
  BusCreator/1 -> Out/1
  In/1 -> Demux/1

== system generic_src/CarMaker/IPG Vehicle/PowerTrain/PTControl Example/PTControl_In/CreateBus PTC MotorIn3 ==
  In : Inport
  BusCreator : BusCreator  Inputs=9
  Demux : Demux  Outputs=9
      settings: DisplayOption=none
  Out : Outport  VectorParamsAs1DForOutWhenUnconnected=off
  wires:
  Demux/9 -> BusCreator/9  "PTC MotorIn3 i_M2W_RR"
  Demux/8 -> BusCreator/8  "PTC MotorIn3 i_M2W_RL"
  Demux/7 -> BusCreator/7  "PTC MotorIn3 i_M2W_FR"
  Demux/6 -> BusCreator/6  "PTC MotorIn3 i_M2W_FL"
  Demux/5 -> BusCreator/5  "PTC MotorIn3 PwrElec"
  Demux/4 -> BusCreator/4  "PTC MotorIn3 TrqGen_max"
  Demux/3 -> BusCreator/3  "PTC MotorIn3 TrqMot_max"
  Demux/2 -> BusCreator/2  "PTC MotorIn3 Trq"
  Demux/1 -> BusCreator/1  "PTC MotorIn3 rotv"
  BusCreator/1 -> Out/1
  In/1 -> Demux/1

== system generic_src/CarMaker/IPG Vehicle/PowerTrain/PTControl Example/PTControl_In/CreateBus PTC MotorIn4 ==
  In : Inport
  BusCreator : BusCreator  Inputs=9
  Demux : Demux  Outputs=9
      settings: DisplayOption=none
  Out : Outport  VectorParamsAs1DForOutWhenUnconnected=off
  wires:
  Demux/9 -> BusCreator/9  "PTC MotorIn4 i_M2W_RR"
  Demux/8 -> BusCreator/8  "PTC MotorIn4 i_M2W_RL"
  Demux/7 -> BusCreator/7  "PTC MotorIn4 i_M2W_FR"
  Demux/6 -> BusCreator/6  "PTC MotorIn4 i_M2W_FL"
  Demux/5 -> BusCreator/5  "PTC MotorIn4 PwrElec"
  Demux/4 -> BusCreator/4  "PTC MotorIn4 TrqGen_max"
  Demux/3 -> BusCreator/3  "PTC MotorIn4 TrqMot_max"
  Demux/2 -> BusCreator/2  "PTC MotorIn4 Trq"
  Demux/1 -> BusCreator/1  "PTC MotorIn4 rotv"
  BusCreator/1 -> Out/1
  In/1 -> Demux/1

== system generic_src/CarMaker/IPG Vehicle/PowerTrain/PTControl Example/PTControl_In/CreateBus PTC MotorIn5 ==
  In : Inport
  BusCreator : BusCreator  Inputs=9
  Demux : Demux  Outputs=9
      settings: DisplayOption=none
  Out : Outport  VectorParamsAs1DForOutWhenUnconnected=off
  wires:
  Demux/9 -> BusCreator/9  "PTC MotorIn5 i_M2W_RR"
  Demux/8 -> BusCreator/8  "PTC MotorIn5 i_M2W_RL"
  Demux/7 -> BusCreator/7  "PTC MotorIn5 i_M2W_FR"
  Demux/6 -> BusCreator/6  "PTC MotorIn5 i_M2W_FL"
  Demux/5 -> BusCreator/5  "PTC MotorIn5 PwrElec"
  Demux/4 -> BusCreator/4  "PTC MotorIn5 TrqGen_max"
  Demux/3 -> BusCreator/3  "PTC MotorIn5 TrqMot_max"
  Demux/2 -> BusCreator/2  "PTC MotorIn5 Trq"
  Demux/1 -> BusCreator/1  "PTC MotorIn5 rotv"
  BusCreator/1 -> Out/1
  In/1 -> Demux/1

== system generic_src/CarMaker/IPG Vehicle/PowerTrain/PTControl Example/PTControl_In/CreateBus PTC MotorIn6 ==
  In : Inport
  BusCreator : BusCreator  Inputs=9
  Demux : Demux  Outputs=9
      settings: DisplayOption=none
  Out : Outport  VectorParamsAs1DForOutWhenUnconnected=off
  wires:
  Demux/9 -> BusCreator/9  "PTC MotorIn6 i_M2W_RR"
  Demux/8 -> BusCreator/8  "PTC MotorIn6 i_M2W_RL"
  Demux/7 -> BusCreator/7  "PTC MotorIn6 i_M2W_FR"
  Demux/6 -> BusCreator/6  "PTC MotorIn6 i_M2W_FL"
  Demux/5 -> BusCreator/5  "PTC MotorIn6 PwrElec"
  Demux/4 -> BusCreator/4  "PTC MotorIn6 TrqGen_max"
  Demux/3 -> BusCreator/3  "PTC MotorIn6 TrqMot_max"
  Demux/2 -> BusCreator/2  "PTC MotorIn6 Trq"
  Demux/1 -> BusCreator/1  "PTC MotorIn6 rotv"
  BusCreator/1 -> Out/1
  In/1 -> Demux/1

== system generic_src/CarMaker/IPG Vehicle/PowerTrain/PTControl Example/PTControl_In/CreateBus PTC MotorIn7 ==
  In : Inport
  BusCreator : BusCreator  Inputs=9
  Demux : Demux  Outputs=9
      settings: DisplayOption=none
  Out : Outport  VectorParamsAs1DForOutWhenUnconnected=off
  wires:
  Demux/9 -> BusCreator/9  "PTC MotorIn7 i_M2W_RR"
  Demux/8 -> BusCreator/8  "PTC MotorIn7 i_M2W_RL"
  Demux/7 -> BusCreator/7  "PTC MotorIn7 i_M2W_FR"
  Demux/6 -> BusCreator/6  "PTC MotorIn7 i_M2W_FL"
  Demux/5 -> BusCreator/5  "PTC MotorIn7 PwrElec"
  Demux/4 -> BusCreator/4  "PTC MotorIn7 TrqGen_max"
  Demux/3 -> BusCreator/3  "PTC MotorIn7 TrqMot_max"
  Demux/2 -> BusCreator/2  "PTC MotorIn7 Trq"
  Demux/1 -> BusCreator/1  "PTC MotorIn7 rotv"
  BusCreator/1 -> Out/1
  In/1 -> Demux/1

== system generic_src/CarMaker/IPG Vehicle/PowerTrain/PTControl Example/PTControl_In/CreateBus PTC MotorIn8 ==
  In : Inport
  BusCreator : BusCreator  Inputs=9
  Demux : Demux  Outputs=9
      settings: DisplayOption=none
  Out : Outport  VectorParamsAs1DForOutWhenUnconnected=off
  wires:
  Demux/9 -> BusCreator/9  "PTC MotorIn8 i_M2W_RR"
  Demux/8 -> BusCreator/8  "PTC MotorIn8 i_M2W_RL"
  Demux/7 -> BusCreator/7  "PTC MotorIn8 i_M2W_FR"
  Demux/6 -> BusCreator/6  "PTC MotorIn8 i_M2W_FL"
  Demux/5 -> BusCreator/5  "PTC MotorIn8 PwrElec"
  Demux/4 -> BusCreator/4  "PTC MotorIn8 TrqGen_max"
  Demux/3 -> BusCreator/3  "PTC MotorIn8 TrqMot_max"
  Demux/2 -> BusCreator/2  "PTC MotorIn8 Trq"
  Demux/1 -> BusCreator/1  "PTC MotorIn8 rotv"
  BusCreator/1 -> Out/1
  In/1 -> Demux/1

== system generic_src/CarMaker/IPG Vehicle/PowerTrain/PTControl Example/PTControl_In/CreateBus PTC MotorIn9 ==
  In : Inport
  BusCreator : BusCreator  Inputs=9
  Demux : Demux  Outputs=9
      settings: DisplayOption=none
  Out : Outport  VectorParamsAs1DForOutWhenUnconnected=off
  wires:
  Demux/9 -> BusCreator/9  "PTC MotorIn9 i_M2W_RR"
  Demux/8 -> BusCreator/8  "PTC MotorIn9 i_M2W_RL"
  Demux/7 -> BusCreator/7  "PTC MotorIn9 i_M2W_FR"
  Demux/6 -> BusCreator/6  "PTC MotorIn9 i_M2W_FL"
  Demux/5 -> BusCreator/5  "PTC MotorIn9 PwrElec"
  Demux/4 -> BusCreator/4  "PTC MotorIn9 TrqGen_max"
  Demux/3 -> BusCreator/3  "PTC MotorIn9 TrqMot_max"
  Demux/2 -> BusCreator/2  "PTC MotorIn9 Trq"
  Demux/1 -> BusCreator/1  "PTC MotorIn9 rotv"
  BusCreator/1 -> Out/1
  In/1 -> Demux/1

== system generic_src/CarMaker/IPG Vehicle/PowerTrain/PTControl Example/PTControl_In/CreateBus PTC PwrSupplyIn ==
  In : Inport
  BusCreator : BusCreator  Inputs=12
  Demux : Demux  Outputs=12
      settings: DisplayOption=none
  Out : Outport  VectorParamsAs1DForOutWhenUnconnected=off
  wires:
  Demux/12 -> BusCreator/12  "PTC PwrSupplyIn Eta_HV1toHV2"
  Demux/11 -> BusCreator/11  "PTC PwrSupplyIn Eta_HV1toLV"
  Demux/10 -> BusCreator/10  "PTC PwrSupplyIn Pwr_HV1toHV2_max"
  Demux/9 -> BusCreator/9  "PTC PwrSupplyIn Pwr_HV1toLV_max"
  Demux/8 -> BusCreator/8  "PTC PwrSupplyIn Pwr_HV1toHV2"
  Demux/7 -> BusCreator/7  "PTC PwrSupplyIn Pwr_HV1toLV"
  Demux/6 -> BusCreator/6  "PTC PwrSupplyIn Voltage_HV2"
  Demux/5 -> BusCreator/5  "PTC PwrSupplyIn Voltage_HV1"
  Demux/4 -> BusCreator/4  "PTC PwrSupplyIn Voltage_LV"
  Demux/3 -> BusCreator/3  "PTC PwrSupplyIn Pwr_HV2"
  Demux/2 -> BusCreator/2  "PTC PwrSupplyIn Pwr_HV1"
  Demux/1 -> BusCreator/1  "PTC PwrSupplyIn Pwr_LV"
  BusCreator/1 -> Out/1
  In/1 -> Demux/1

== system generic_src/CarMaker/IPG Vehicle/PowerTrain/PTControl Example/PTControl_In/CreateBus PTC Vehicle Ctrl ==
  In : Inport
  BusCreator : BusCreator  Inputs=8
  Demux : Demux  Outputs=8
      settings: DisplayOption=none
  Out : Outport  VectorParamsAs1DForOutWhenUnconnected=off
  wires:
  Demux/8 -> BusCreator/8  "PTC Velocity"
  Demux/7 -> BusCreator/7  "PTC Brake"
  Demux/6 -> BusCreator/6  "PTC Gas"
  Demux/5 -> BusCreator/5  "PTC Clutch"
  Demux/4 -> BusCreator/4  "PTC GearNoTrg"
  Demux/3 -> BusCreator/3  "PTC SelectorCtrl"
  Demux/2 -> BusCreator/2  "PTC SST"
  Demux/1 -> BusCreator/1  "PTC Key"
  BusCreator/1 -> Out/1
  In/1 -> Demux/1

== system generic_src/CarMaker/IPG Vehicle/PowerTrain/PTControl Example/PTControl_In/CreateBus PTC WheelIn ==
  In : Inport
  BusCreator : BusCreator  Inputs=4
  Demux : Demux
      settings: DisplayOption=none
  Out : Outport  VectorParamsAs1DForOutWhenUnconnected=off
  wires:
  Demux/4 -> BusCreator/4  "PTC WheelIn_RR Trq_BrakeReg_trg"
  Demux/3 -> BusCreator/3  "PTC WheelIn_RL Trq_BrakeReg_trg"
  Demux/2 -> BusCreator/2  "PTC WheelIn_FR Trq_BrakeReg_trg"
  Demux/1 -> BusCreator/1  "PTC WheelIn_FL Trq_BrakeReg_trg"
  BusCreator/1 -> Out/1
  In/1 -> Demux/1

== system generic_src/CarMaker/IPG Vehicle/PowerTrain/PTControl Example/PTControl_In/CreateBus PTC_Cfg BatteryHV ==
  In : Inport
  BusCreator : BusCreator  Inputs=6
  Demux : Demux  Outputs=6
      settings: DisplayOption=none
  Out : Outport  VectorParamsAs1DForOutWhenUnconnected=off
  wires:
  Demux/2 -> BusCreator/2  "PTC_Cfg BattHV SOC_max"
  Demux/5 -> BusCreator/5  "PTC_Cfg BattHV Temp_init"
  Demux/6 -> BusCreator/6  "PTC_Cfg BattHV TempCool_init"
  Demux/1 -> BusCreator/1  "PTC_Cfg BattHV SOC_min"
  BusCreator/1 -> Out/1
  Demux/4 -> BusCreator/4  "PTC_Cfg BattHV Voltage"
  In/1 -> Demux/1
  Demux/3 -> BusCreator/3  "PTC_Cfg BattHV Capacity"

== system generic_src/CarMaker/IPG Vehicle/PowerTrain/PTControl Example/PTControl_In/CreateBus PTC_Cfg BatteryLV ==
  In : Inport
  BusCreator : BusCreator  Inputs=6
  Demux : Demux  Outputs=6
      settings: DisplayOption=none
  Out : Outport  VectorParamsAs1DForOutWhenUnconnected=off
  wires:
  Demux/3 -> BusCreator/3  "PTC_Cfg BattLV Capacity"
  In/1 -> Demux/1
  Demux/4 -> BusCreator/4  "PTC_Cfg BattLV Voltage"
  BusCreator/1 -> Out/1
  Demux/1 -> BusCreator/1  "PTC_Cfg BattLV SOC_min"
  Demux/6 -> BusCreator/6  "PTC_Cfg BattLV TempCool_init"
  Demux/5 -> BusCreator/5  "PTC_Cfg BattLV Temp_init"
  Demux/2 -> BusCreator/2  "PTC_Cfg BattLV SOC_max"

== system generic_src/CarMaker/IPG Vehicle/PowerTrain/PTControl Example/PTControl_In/CreateBus PTC_Cfg Engine ==
  In : Inport
  BusCreator : BusCreator  Inputs=4
  Demux : Demux
      settings: DisplayOption=none
  Out : Outport  VectorParamsAs1DForOutWhenUnconnected=off
  wires:
  Demux/4 -> BusCreator/4  "PTC_Cfg Engine rotv_opt"
  Demux/3 -> BusCreator/3  "PTC_Cfg Engine rotv_idle"
  Demux/2 -> BusCreator/2  "PTC_Cfg Engine rotv_max"
  Demux/1 -> BusCreator/1  "PTC_Cfg Engine Fuel_l2kWh"
  BusCreator/1 -> Out/1
  In/1 -> Demux/1

== system generic_src/CarMaker/IPG Vehicle/PowerTrain/PTControl Example/PTControl_In/CreateBus PTC_Cfg GearBox0 ==
  In : Inport
  BusCreator : BusCreator  Inputs=38
  Demux : Demux  Outputs=38
      settings: DisplayOption=none
  Out : Outport  VectorParamsAs1DForOutWhenUnconnected=off
  wires:
  Demux/38 -> BusCreator/38  "PTC_Cfg GearBox0 iBGear16"
  Demux/37 -> BusCreator/37  "PTC_Cfg GearBox0 iBGear15"
  Demux/36 -> BusCreator/36  "PTC_Cfg GearBox0 iBGear14"
  Demux/35 -> BusCreator/35  "PTC_Cfg GearBox0 iBGear13"
  Demux/34 -> BusCreator/34  "PTC_Cfg GearBox0 iBGear12"
  Demux/33 -> BusCreator/33  "PTC_Cfg GearBox0 iBGear11"
  Demux/32 -> BusCreator/32  "PTC_Cfg GearBox0 iBGear10"
  Demux/31 -> BusCreator/31  "PTC_Cfg GearBox0 iBGear9"
  Demux/30 -> BusCreator/30  "PTC_Cfg GearBox0 iBGear8"
  Demux/29 -> BusCreator/29  "PTC_Cfg GearBox0 iBGear7"
  Demux/28 -> BusCreator/28  "PTC_Cfg GearBox0 iBGear6"
  Demux/27 -> BusCreator/27  "PTC_Cfg GearBox0 iBGear5"
  Demux/26 -> BusCreator/26  "PTC_Cfg GearBox0 iBGear4"
  Demux/25 -> BusCreator/25  "PTC_Cfg GearBox0 iBGear3"
  Demux/24 -> BusCreator/24  "PTC_Cfg GearBox0 iBGear2"
  Demux/23 -> BusCreator/23  "PTC_Cfg GearBox0 iBGear1"
  Demux/22 -> BusCreator/22  "PTC_Cfg GearBox0 iBGear0"
  Demux/21 -> BusCreator/21  "PTC_Cfg GearBox0 nBGears"
  Demux/20 -> BusCreator/20  "PTC_Cfg GearBox0 iFGear16"
  Demux/19 -> BusCreator/19  "PTC_Cfg GearBox0 iFGear15"
  Demux/18 -> BusCreator/18  "PTC_Cfg GearBox0 iFGear14"
  Demux/17 -> BusCreator/17  "PTC_Cfg GearBox0 iFGear13"
  Demux/16 -> BusCreator/16  "PTC_Cfg GearBox0 iFGear12"
  Demux/15 -> BusCreator/15  "PTC_Cfg GearBox0 iFGear11"
  Demux/14 -> BusCreator/14  "PTC_Cfg GearBox0 iFGear10"
  Demux/13 -> BusCreator/13  "PTC_Cfg GearBox0 iFGear9"
  Demux/12 -> BusCreator/12  "PTC_Cfg GearBox0 iFGear8"
  Demux/11 -> BusCreator/11  "PTC_Cfg GearBox0 iFGear7"
  Demux/10 -> BusCreator/10  "PTC_Cfg GearBox0 iFGear6"
  Demux/9 -> BusCreator/9  "PTC_Cfg GearBox0 iFGear5"
  Demux/8 -> BusCreator/8  "PTC_Cfg GearBox0 iFGear4"
  Demux/7 -> BusCreator/7  "PTC_Cfg GearBox0 iFGear3"
  Demux/6 -> BusCreator/6  "PTC_Cfg GearBox0 iFGear2"
  Demux/5 -> BusCreator/5  "PTC_Cfg GearBox0 iFGear1"
  Demux/4 -> BusCreator/4  "PTC_Cfg GearBox0 iFGear0"
  Demux/3 -> BusCreator/3  "PTC_Cfg GearBox0 nFGears"
  Demux/2 -> BusCreator/2  "PTC_Cfg GearBox0 ClKind"
  Demux/1 -> BusCreator/1  "PTC_Cfg GearBox0 GBKind"
  BusCreator/1 -> Out/1
  In/1 -> Demux/1

== system generic_src/CarMaker/IPG Vehicle/PowerTrain/PTControl Example/PTControl_In/CreateBus PTC_Cfg GearBox1 ==
  In : Inport
  BusCreator : BusCreator  Inputs=38
  Demux : Demux  Outputs=38
      settings: DisplayOption=none
  Out : Outport  VectorParamsAs1DForOutWhenUnconnected=off
  wires:
  Demux/38 -> BusCreator/38  "PTC_Cfg GearBox1 iBGear16"
  Demux/37 -> BusCreator/37  "PTC_Cfg GearBox1 iBGear15"
  Demux/36 -> BusCreator/36  "PTC_Cfg GearBox1 iBGear14"
  Demux/35 -> BusCreator/35  "PTC_Cfg GearBox1 iBGear13"
  Demux/34 -> BusCreator/34  "PTC_Cfg GearBox1 iBGear12"
  Demux/33 -> BusCreator/33  "PTC_Cfg GearBox1 iBGear11"
  Demux/32 -> BusCreator/32  "PTC_Cfg GearBox1 iBGear10"
  Demux/31 -> BusCreator/31  "PTC_Cfg GearBox1 iBGear9"
  Demux/30 -> BusCreator/30  "PTC_Cfg GearBox1 iBGear8"
  Demux/29 -> BusCreator/29  "PTC_Cfg GearBox1 iBGear7"
  Demux/28 -> BusCreator/28  "PTC_Cfg GearBox1 iBGear6"
  Demux/27 -> BusCreator/27  "PTC_Cfg GearBox1 iBGear5"
  Demux/26 -> BusCreator/26  "PTC_Cfg GearBox1 iBGear4"
  Demux/25 -> BusCreator/25  "PTC_Cfg GearBox1 iBGear3"
  Demux/24 -> BusCreator/24  "PTC_Cfg GearBox1 iBGear2"
  Demux/23 -> BusCreator/23  "PTC_Cfg GearBox1 iBGear1"
  Demux/22 -> BusCreator/22  "PTC_Cfg GearBox1 iBGear0"
  Demux/21 -> BusCreator/21  "PTC_Cfg GearBox1 nBGears"
  Demux/20 -> BusCreator/20  "PTC_Cfg GearBox1 iFGear16"
  Demux/19 -> BusCreator/19  "PTC_Cfg GearBox1 iFGear15"
  Demux/18 -> BusCreator/18  "PTC_Cfg GearBox1 iFGear14"
  Demux/17 -> BusCreator/17  "PTC_Cfg GearBox1 iFGear13"
  Demux/16 -> BusCreator/16  "PTC_Cfg GearBox1 iFGear12"
  Demux/15 -> BusCreator/15  "PTC_Cfg GearBox1 iFGear11"
  Demux/14 -> BusCreator/14  "PTC_Cfg GearBox1 iFGear10"
  Demux/13 -> BusCreator/13  "PTC_Cfg GearBox1 iFGear9"
  Demux/12 -> BusCreator/12  "PTC_Cfg GearBox1 iFGear8"
  Demux/11 -> BusCreator/11  "PTC_Cfg GearBox1 iFGear7"
  Demux/10 -> BusCreator/10  "PTC_Cfg GearBox1 iFGear6"
  Demux/9 -> BusCreator/9  "PTC_Cfg GearBox1 iFGear5"
  Demux/8 -> BusCreator/8  "PTC_Cfg GearBox1 iFGear4"
  Demux/7 -> BusCreator/7  "PTC_Cfg GearBox1 iFGear3"
  Demux/6 -> BusCreator/6  "PTC_Cfg GearBox1 iFGear2"
  Demux/5 -> BusCreator/5  "PTC_Cfg GearBox1 iFGear1"
  Demux/4 -> BusCreator/4  "PTC_Cfg GearBox1 iFGear0"
  Demux/3 -> BusCreator/3  "PTC_Cfg GearBox1 nFGears"
  Demux/2 -> BusCreator/2  "PTC_Cfg GearBox1 ClKind"
  Demux/1 -> BusCreator/1  "PTC_Cfg GearBox1 GBKind"
  BusCreator/1 -> Out/1
  In/1 -> Demux/1
